simulink model "BoostPFC"  (R2023b)
settings: Solver=VariableStepAuto  StartTime=0.0  StopTime=1.3  RelTol=1e-3
libraries: spsDiodeLib x16, spsSeriesRLCBranchLib x8, spsVoltageMeasurementLib x5, spsCurrentMeasurementLib x4, spsACVoltageSourceLib x3, slpidlib x2, spsMosfetLib x1, spsPWMGeneratorDCDCLib x1, sps_lib x1
settings Model: Creator=yigex  LastModifiedBy=yigex

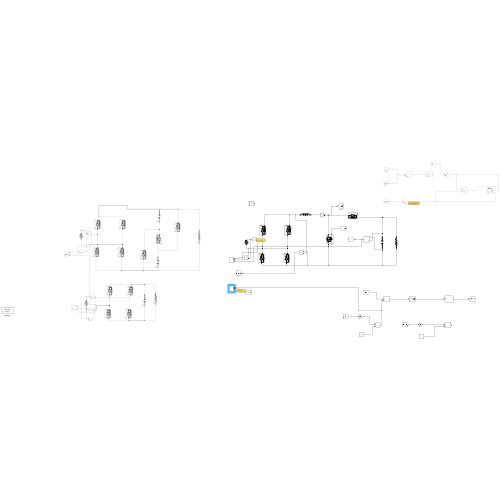
[thumbnail: Simulink's stored preview of the top-level diagram]
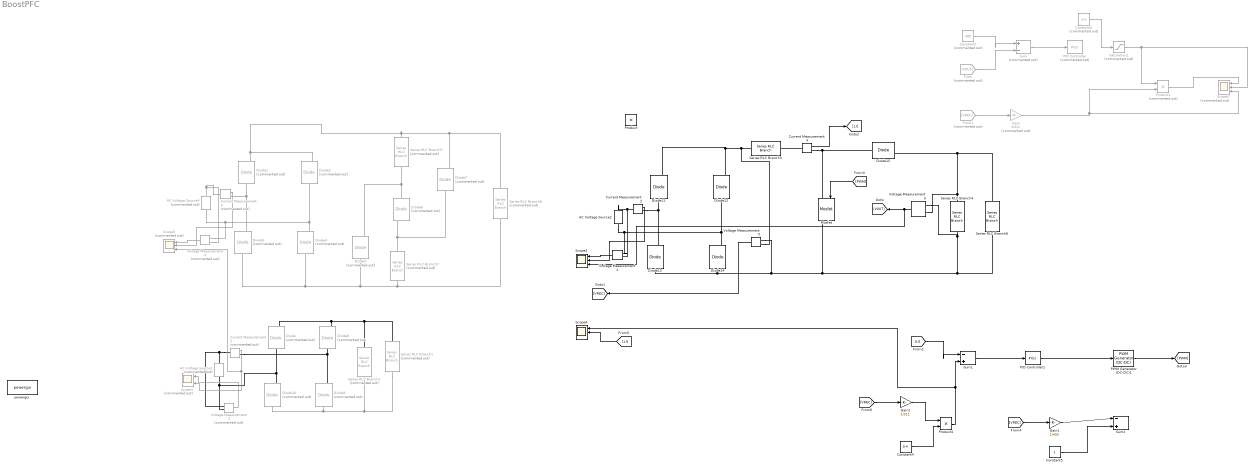
== system BoostPFC ==
  AC Voltage Source1 : spsACVoltageSourceLib/AC Voltage Source  Commented=on  Amplitude=310  Phase=0  Frequency=60  SampleTime=0  Measurements=None  BusType=swing  Pref=10e3  Qref=0  Qmin=-inf  Qmax=+inf
  AC Voltage Source2 : spsACVoltageSourceLib/AC Voltage Source  Amplitude=311  Phase=0  Frequency=50  SampleTime=0  Measurements=None  BusType=swing  Pref=10e3  Qref=0  Qmin=-inf  Qmax=+inf
  AC Voltage Source4 : spsACVoltageSourceLib/AC Voltage Source  Commented=on  Amplitude=310  Phase=0  Frequency=60  SampleTime=0  Measurements=None  BusType=swing  Pref=10e3  Qref=0  Qmin=-inf  Qmax=+inf
  Constant1 : Constant  Commented=on  Value=400
  Constant3 : Constant  Commented=on  Value=0.4
  Constant4 : Constant  Value=0.4
  Constant5 : Constant
  Current Measurement1 : spsCurrentMeasurementLib/Current Measurement  Commented=on  PhasorSimulation=off  OutputType=Complex  PSBequivalent=0
  Current Measurement2 : spsCurrentMeasurementLib/Current Measurement  PhasorSimulation=off  OutputType=Complex  PSBequivalent=0
  Current Measurement3 : spsCurrentMeasurementLib/Current Measurement  PhasorSimulation=off  OutputType=Complex  PSBequivalent=0
  Current Measurement4 : spsCurrentMeasurementLib/Current Measurement  Commented=on  PhasorSimulation=off  OutputType=Complex  PSBequivalent=0
  Diode{,1..10} (11 alike) : spsDiodeLib/Diode  Commented=on  Ron=0.001  Lon=0  Vf=0.8  IC=0  UseSnubber=0  Rs=500  Cs=250e-9  Measurements=on
  Diode{11..15} (5 alike) : spsDiodeLib/Diode  Ron=0.001  Lon=0  Vf=0.8  IC=0  UseSnubber=0  Rs=500  Cs=250e-9  Measurements=on
  From : From  Commented=on  GotoTag=VOUT
  From1 : From  Commented=on  GotoTag=VREC
  Gain : Gain  Commented=on  Gain=1/311
  Gain1 : Gain  Gain=1/400
  Gain2 : Gain  Gain=1/311
  Mosfet : spsMosfetLib/Mosfet  Ron=0.1  Lon=0  Rd=0.01  Vfd=0  IC=0  Rs=1e5  Cs=inf  Measurements=on
  PID Controller : slpidlib/PID Controller  Commented=on  Controller=PI  Form=Parallel  TimeDomain=Continuous-time  UseExternalTs=off  SampleTime=-1  IntegratorMethod=Forward Euler  FilterMethod=Forward Euler  ControllerParametersSource=internal  P=0.02  I=2  UseKiTs=off  D=0  N=100  UseFilter=on  TunerSelectOption=Transfer Function Based (PID Tuner App)  InitialConditionSource=internal  InitialConditionForIntegrator=0  InitialConditionForFilter=0  DifferentiatorICPrevScaledInput=0  ExternalReset=none  TrackingMode=off  Kt=1  LimitOutput=off  SatLimitsSource=internal  UpperSaturationLimit=inf  LowerSaturationLimit=-inf  LinearizeAsGain=on  AntiWindupMode=none  Kb=1  LimitIntegrator=off  UpperIntegratorSaturationLimit=inf  LowerIntegratorSaturationLimit=-inf  POutMin=[]  POutMax=[]  IOutMin=[]  IOutMax=[]  DOutMin=[]  DOutMax=[]  NOutMin=[]  NOutMax=[]  SumOutMin=[]  SumOutMax=[]  SaturationOutMin=[]  SaturationOutMax=[]  PParamMin=[]  PParamMax=[]  IParamMin=[]  IParamMax=[]  DParamMin=[]  DParamMax=[]  NParamMin=[]  NParamMax=[]  KbParamMin=[]  KbParamMax=[]  KtParamMin=[]  KtParamMax=[]  KbOutMin=[]  KbOutMax=[]  KtOutMin=[]  KtOutMax=[]  IntegratorOutMin=[]  IntegratorOutMax=[]  FilterOutMin=[]  FilterOutMax=[]  SumI1OutMin=[]  SumI1OutMax=[]  SumI2OutMin=[]  SumI2OutMax=[]  SumI3OutMin=[]  SumI3OutMax=[]  SumI4OutMin=[]  SumI4OutMax=[]  SumDOutMin=[]  SumDOutMax=[]  DifferentiatorOutMin=[]  DifferentiatorOutMax=[]  FilterDiffOutCoefMin=[]  FilterDiffOutCoefMax=[]  ReciprocalOutMin=[]  ReciprocalOutMax=[]  SumDenOutMin=[]  SumDenOutMax=[]  SumNumOutMin=[]  SumNumOutMax=[]  DivideOutMin=[]  DivideOutMax=[]  UdiffTsProdOutMin=[]  UdiffTsProdOutMax=[]  NTsProdOutMin=[]  NTsProdOutMax=[]  UintegralTsProdOutMin=[]  UintegralTsProdOutMax=[]  UngainTsProdOutMin=[]  UngainTsProdOutMax=[]  ClampingZeroOutDataTypeStr=Inherit: Inherit via back propagation  ClampingZeroOutMin=[]  ClampingZeroOutMax=[]  FilterDenConstantOutDataTypeStr=Inherit: Inherit via back propagation  FilterDenConstantOutMin=[]  FilterDenConstantOutMax=[]  PCopyOutDataTypeStr=Inherit: Inherit via back propagation  PCopyOutMin=[]  PCopyOutMax=[]  NCopyOutDataTypeStr=Inherit: Inherit via back propagation  NCopyOutMin=[]  NCopyOutMax=[]  IntegratorContinuousStateAttributes=''  IntegratorStateMustResolveToSignalObject=off  IntegratorRTWStateStorageClass=Auto  FilterContinuousStateAttributes=''  FilterStateMustResolveToSignalObject=off  FilterRTWStateStorageClass=Auto  ParallelPVariant=InternalParameters  IdealPVariant=Disabled  IVariant=InternalParameters  DVariant=Disabled  IntegratorVariant=Continuous  SatVariant=Disabled  AWVariant=Passthrough  PCopyVariant=Disabled  TRVariant=Disabled  FdbkBlocksVariant=Forward  IdealPFdbkVariant=Disabled  SatFdbkVariant=Disabled  DerivativeFilterVariant=Disabled  NVariant=Disabled  NCopyVariant=Disabled_SignalSpec  FilterICVariant=Disabled  IntegratorICVariant=InternalICs  ExternalResetVariant=Disabled  TRSumVariant=Passthrough  SumFdbkVariant=Disabled  SumVariant=Sum_PI  TsampFilterVariant=InternalTs  TsampNgainVariant=Passthrough  TsampIntegralVariant=Disabled_SignalSpec  ExternalSaturationOutDataTypeStr=Inherit: Same as second input
  PID Controller1 : slpidlib/PID Controller  Controller=PI  Form=Parallel  TimeDomain=Continuous-time  UseExternalTs=off  SampleTime=-1  IntegratorMethod=Forward Euler  FilterMethod=Forward Euler  ControllerParametersSource=internal  P=0.05  I=50  UseKiTs=off  D=0  N=100  UseFilter=on  TunerSelectOption=Transfer Function Based (PID Tuner App)  InitialConditionSource=internal  InitialConditionForIntegrator=0  InitialConditionForFilter=0  DifferentiatorICPrevScaledInput=0  ExternalReset=none  TrackingMode=off  Kt=1  LimitOutput=on  SatLimitsSource=internal  UpperSaturationLimit=0.9  LowerSaturationLimit=0  LinearizeAsGain=on  AntiWindupMode=clamping  Kb=1  LimitIntegrator=off  UpperIntegratorSaturationLimit=inf  LowerIntegratorSaturationLimit=-inf  POutMin=[]  POutMax=[]  IOutMin=[]  IOutMax=[]  DOutMin=[]  DOutMax=[]  NOutMin=[]  NOutMax=[]  SumOutMin=[]  SumOutMax=[]  SaturationOutMin=[]  SaturationOutMax=[]  PParamMin=[]  PParamMax=[]  IParamMin=[]  IParamMax=[]  DParamMin=[]  DParamMax=[]  NParamMin=[]  NParamMax=[]  KbParamMin=[]  KbParamMax=[]  KtParamMin=[]  KtParamMax=[]  KbOutMin=[]  KbOutMax=[]  KtOutMin=[]  KtOutMax=[]  IntegratorOutMin=[]  IntegratorOutMax=[]  FilterOutMin=[]  FilterOutMax=[]  SumI1OutMin=[]  SumI1OutMax=[]  SumI2OutMin=[]  SumI2OutMax=[]  SumI3OutMin=[]  SumI3OutMax=[]  SumI4OutMin=[]  SumI4OutMax=[]  SumDOutMin=[]  SumDOutMax=[]  DifferentiatorOutMin=[]  DifferentiatorOutMax=[]  FilterDiffOutCoefMin=[]  FilterDiffOutCoefMax=[]  ReciprocalOutMin=[]  ReciprocalOutMax=[]  SumDenOutMin=[]  SumDenOutMax=[]  SumNumOutMin=[]  SumNumOutMax=[]  DivideOutMin=[]  DivideOutMax=[]  UdiffTsProdOutMin=[]  UdiffTsProdOutMax=[]  NTsProdOutMin=[]  NTsProdOutMax=[]  UintegralTsProdOutMin=[]  UintegralTsProdOutMax=[]  UngainTsProdOutMin=[]  UngainTsProdOutMax=[]  ClampingZeroOutDataTypeStr=Inherit: Inherit via back propagation  ClampingZeroOutMin=[]  ClampingZeroOutMax=[]  FilterDenConstantOutDataTypeStr=Inherit: Inherit via back propagation  FilterDenConstantOutMin=[]  FilterDenConstantOutMax=[]  PCopyOutDataTypeStr=Inherit: Inherit via back propagation  PCopyOutMin=[]  PCopyOutMax=[]  NCopyOutDataTypeStr=Inherit: Inherit via back propagation  NCopyOutMin=[]  NCopyOutMax=[]  IntegratorContinuousStateAttributes=''  IntegratorStateMustResolveToSignalObject=off  IntegratorRTWStateStorageClass=Auto  FilterContinuousStateAttributes=''  FilterStateMustResolveToSignalObject=off  FilterRTWStateStorageClass=Auto  ParallelPVariant=InternalParameters  IdealPVariant=Disabled  IVariant=InternalParameters  DVariant=Disabled  IntegratorVariant=Continuous  SatVariant=Enabled  AWVariant=ContClampingParallel  PCopyVariant=Disabled  TRVariant=Disabled  FdbkBlocksVariant=Forward  IdealPFdbkVariant=Disabled  SatFdbkVariant=Disabled  DerivativeFilterVariant=Disabled  NVariant=Disabled  NCopyVariant=Disabled_SignalSpec  FilterICVariant=Disabled  IntegratorICVariant=InternalICs  ExternalResetVariant=Disabled  TRSumVariant=Passthrough  SumFdbkVariant=Disabled  SumVariant=Sum_PI  TsampFilterVariant=InternalTs  TsampNgainVariant=Passthrough  TsampIntegralVariant=Disabled_SignalSpec  ExternalSaturationOutDataTypeStr=Inherit: Same as second input
  PWM Generator (DC-DC)1 : spsPWMGeneratorDCDCLib/PWM Generator (DC-DC)  Fsw=500000  Ts=0
  Product : Product
  Product1 : Product  Commented=on
  Product2 : Product
  Saturation1 : Saturate  Commented=on  UpperLimit=2  LowerLimit=0
  Scope1 : Scope  Commented=on  NumInputPorts=2
  Scope2 : Scope  NumInputPorts=3
  Scope3 : Scope  Commented=on  NumInputPorts=3
  Scope4 : Scope  NumInputPorts=3
  Scope5 : Scope  Commented=on  NumInputPorts=3
  Series RLC Branch1 : spsSeriesRLCBranchLib/Series RLC Branch  Commented=on  LConnTagsString=__new0  RConnTagsString=__new0  BranchType=R  Resistance=20  Inductance=220e-3  SetiL0=off  InitialCurrent=0  Capacitance=220e-6  Setx0=off  InitialVoltage=0  Measurements=None
  Series RLC Branch2 : spsSeriesRLCBranchLib/Series RLC Branch  Commented=on  LConnTagsString=__new0  RConnTagsString=__new0  BranchType=C  Resistance=10  Inductance=220e-3  SetiL0=off  InitialCurrent=0  Capacitance=220e-6  Setx0=off  InitialVoltage=0  Measurements=None
  Series RLC Branch3 : spsSeriesRLCBranchLib/Series RLC Branch  LConnTagsString=__new0  RConnTagsString=__new0  BranchType=L  Resistance=20  Inductance=10e-3  SetiL0=off  InitialCurrent=0  Capacitance=1e-6  Setx0=off  InitialVoltage=0  Measurements=None
  Series RLC Branch4 : spsSeriesRLCBranchLib/Series RLC Branch  LConnTagsString=__new0  RConnTagsString=__new0  BranchType=C  Resistance=1  Inductance=220e-3  SetiL0=off  InitialCurrent=0  Capacitance=470e-6  Setx0=off  InitialVoltage=0  Measurements=None
  Series RLC Branch5 : spsSeriesRLCBranchLib/Series RLC Branch  Commented=on  LConnTagsString=__new0  RConnTagsString=__new0  BranchType=C  Resistance=1  Inductance=220e-3  SetiL0=off  InitialCurrent=0  Capacitance=220e-6  Setx0=off  InitialVoltage=0  Measurements=None
  Series RLC Branch6 : spsSeriesRLCBranchLib/Series RLC Branch  LConnTagsString=__new0  RConnTagsString=__new0  BranchType=R  Resistance=3000  Inductance=1e-3  SetiL0=off  InitialCurrent=0  Capacitance=1e-6  Setx0=off  InitialVoltage=0  Measurements=None
  Series RLC Branch7 : spsSeriesRLCBranchLib/Series RLC Branch  Commented=on  LConnTagsString=__new0  RConnTagsString=__new0  BranchType=C  Resistance=1  Inductance=220e-3  SetiL0=off  InitialCurrent=0  Capacitance=220e-6  Setx0=off  InitialVoltage=0  Measurements=None
  Series RLC Branch8 : spsSeriesRLCBranchLib/Series RLC Branch  Commented=on  LConnTagsString=__new0  RConnTagsString=__new0  BranchType=R  Resistance=20  Inductance=1e-3  SetiL0=off  InitialCurrent=0  Capacitance=1e-6  Setx0=off  InitialVoltage=0  Measurements=None
  Sum : Sum  Commented=on  Inputs=|+-
  Sum1 : Sum  Inputs=|-+
  Sum2 : Sum  Inputs=|-+
  Voltage Measurement1 : spsVoltageMeasurementLib/Voltage Measurement  Commented=on  PhasorSimulation=off  OutputType=Complex  PSBequivalent=0
  Voltage Measurement2 : spsVoltageMeasurementLib/Voltage Measurement  PhasorSimulation=off  OutputType=Complex  PSBequivalent=0
  Voltage Measurement3 : spsVoltageMeasurementLib/Voltage Measurement  PhasorSimulation=off  OutputType=Complex  PSBequivalent=0
  Voltage Measurement4 : spsVoltageMeasurementLib/Voltage Measurement  Commented=on  PhasorSimulation=off  OutputType=Complex  PSBequivalent=0
  Voltage Measurement5 : spsVoltageMeasurementLib/Voltage Measurement  PhasorSimulation=off  OutputType=Complex  PSBequivalent=0
  powergui : sps_lib/powergui  Priority=1  SimulationMode=Discrete  SampleTime=1e-6  frequency=60  Iterations=50  frequencyindice=50  Pbase=100e6  ErrMax=1e-4  UnitsV=kV  UnitsW=MW  buscounter=0  FunctionMessages=off  echomessages=off  EnableUseOfTLC=off  CurrentSourceSwitches=off  DisableSnubberDevices=off  DisableRonSwitches=off  DisableVfSwitches=off  DisplayEquations=off  AutomaticDiscreteSolvers=off  SolverType=Tustin/Backward Euler (TBE)  Interpol=off  ExternalGateDelay=off  methode=off  Ts=100  x0status=blocks  SPID=on  SwTol=0  HookPort=off  NonlinearTolerance=1e-4  nMaxIteration=100  ContinueOnMaxIteration=off  RestoreLinks=warning  ResistiveCurrentMeasurement=off  Frange=[0:2:500]  Ylog=off  Xlog=on  ShowGrid=off  save=off  variable=ZData  structure=0  ZoomFFT=off  StartTime=0.0  cycles=1  DisplayStyle=1  fundamental=60  FreqAxis=off  MaxFrequency=1000  frequencyindicesteady=1  RmsSteady=1  display=off
  wires:
  Voltage Measurement4/1 -> Scope5/1
  Current Measurement4/1 -> Scope5/2
  Voltage Measurement1/1 -> Scope1/1
  Current Measurement1/1 -> Scope5/3, Scope1/2
  Current Measurement2/1 -> Scope2/2
  Voltage Measurement2/1 -> Scope2/1
  Constant1/1 -> Sum/1
  From/1 -> Sum/2
  Voltage Measurement3/1 -> Scope2/3, [VOUT]
  Sum/1 -> PID Controller/1
  Saturation1/1 -> Scope3/2, Product1/1
  From1/1 -> Gain/1
  Gain/1 -> Scope3/3, Product1/2
  Product1/1 -> Scope3/1
  Constant3/1 -> Saturation1/1
  Current Measurement3/1 -> [LI]
  [LI] -> Sum1/1
  Sum1/1 -> PID Controller1/1
  PID Controller1/1 -> PWM Generator (DC-DC)1/1
  PWM Generator (DC-DC)1/1 -> [PWM]
  [PWM] -> Mosfet/1
  [LI] -> Scope4/2
  [VREC] -> Gain1/1
  Constant5/1 -> Sum2/2
  Gain1/1 -> Sum2/1
  [VREC] -> Gain2/1
  Gain2/1 -> Product2/1
  Constant4/1 -> Product2/2
  Product2/1 -> Scope4/1, Sum1/2
  Voltage Measurement5/1 -> [VREC]
  connections:
  Diode3/RConn1 -- Current Measurement4/RConn1 -- Diode1/LConn1
  Diode4/RConn1 -- Voltage Measurement4/LConn2 -- AC Voltage Source4/LConn1 -- Diode2/LConn1
  Diode1/RConn1 -- Series RLC Branch5/LConn1 -- Series RLC Branch8/LConn1 -- Diode7/RConn1 -- Diode2/RConn1
  Diode3/LConn1 -- Series RLC Branch8/RConn1 -- Series RLC Branch7/RConn1 -- Diode5/LConn1 -- Diode4/LConn1
  Diode6/LConn1 -- Diode5/RConn1 -- Series RLC Branch5/RConn1
  Series RLC Branch7/LConn1 -- Diode7/LConn1 -- Diode6/RConn1
  AC Voltage Source4/RConn1 -- Voltage Measurement4/LConn1 -- Current Measurement4/LConn1
  Current Measurement1/LConn1 -- AC Voltage Source1/RConn1 -- Voltage Measurement1/LConn1
  Diode/LConn1 -- Diode10/RConn1 -- AC Voltage Source1/LConn1 -- Voltage Measurement1/LConn2
  Series RLC Branch1/RConn1 -- Series RLC Branch2/RConn1 -- Diode10/LConn1 -- Diode9/LConn1
  Diode8/LConn1 -- Diode9/RConn1 -- Current Measurement1/RConn1
  Diode8/RConn1 -- Diode/RConn1 -- Series RLC Branch2/LConn1 -- Series RLC Branch1/LConn1
  Current Measurement2/LConn1 -- AC Voltage Source2/RConn1 -- Voltage Measurement2/LConn1
  Diode11/LConn1 -- Current Measurement2/RConn1 -- Diode13/RConn1
  Diode12/LConn1 -- Diode14/RConn1 -- Voltage Measurement2/LConn2 -- AC Voltage Source2/LConn1
  Diode11/RConn1 -- Voltage Measurement5/LConn1 -- Series RLC Branch3/LConn1 -- Diode12/RConn1
  Current Measurement3/LConn1 -- Series RLC Branch3/RConn1
  Current Measurement3/RConn1 -- Diode15/LConn1 -- Mosfet/LConn1
  Mosfet/RConn1 -- Voltage Measurement3/LConn2 -- Series RLC Branch4/RConn1 -- Series RLC Branch6/RConn1 -- Voltage Measurement5/LConn2 -- Diode13/LConn1 -- Diode14/LConn1
  Series RLC Branch4/LConn1 -- Series RLC Branch6/LConn1 -- Diode15/RConn1 -- Voltage Measurement3/LConn1
